simulink model "SPPC"  (R2026a)
settings: Solver=FixedStepDiscrete  StopTime=inf  FixedStep=Ts
model workspace (MATLAB code in the model file):
  | % Defaults for standalone use and code generation, from HPP_parameters.
  | % In HPP.slx the Model block passes p.ctrl.sppc.par as the argument "par".
  | pDefault = HPP_parameters();
  | Ts  = pDefault.ctrl.sppc.Ts;    % [s] fixed sample time
  | par = pDefault.ctrl.sppc.par;   % tunable parameters (model argument)
  | N   = numel(par.share);   % asset instances (fixed per build)
  | clear pDefault
libraries: simulink x5, slpidlib x2, sl_discontinuities x1
Description:
  | SPPC plant controller: WECC REPC_A structure (P control with frequency droop and PI, Q or voltage control with PI, references fed forward), closed loop on the plant feeder into the 33 kV busbar, then dispatch over the N assets by availability. Per unit on the plant rating. Parameters: model argument par (= p.ctrl.sppc.par, from p.pc.sppc).
settings Model: ParameterArgumentNames=par  Creator=kjaer  LastModifiedBy=kjaer

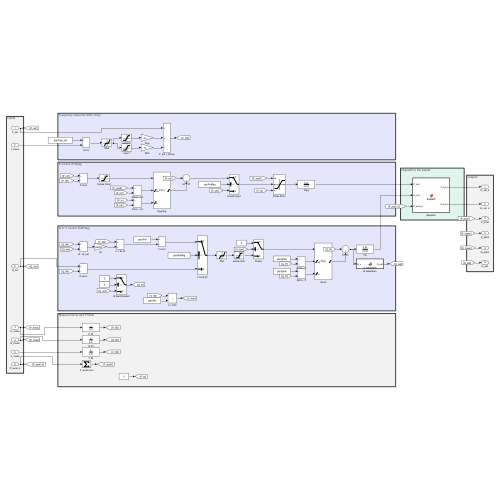
[thumbnail: Simulink's stored preview of the top-level diagram]
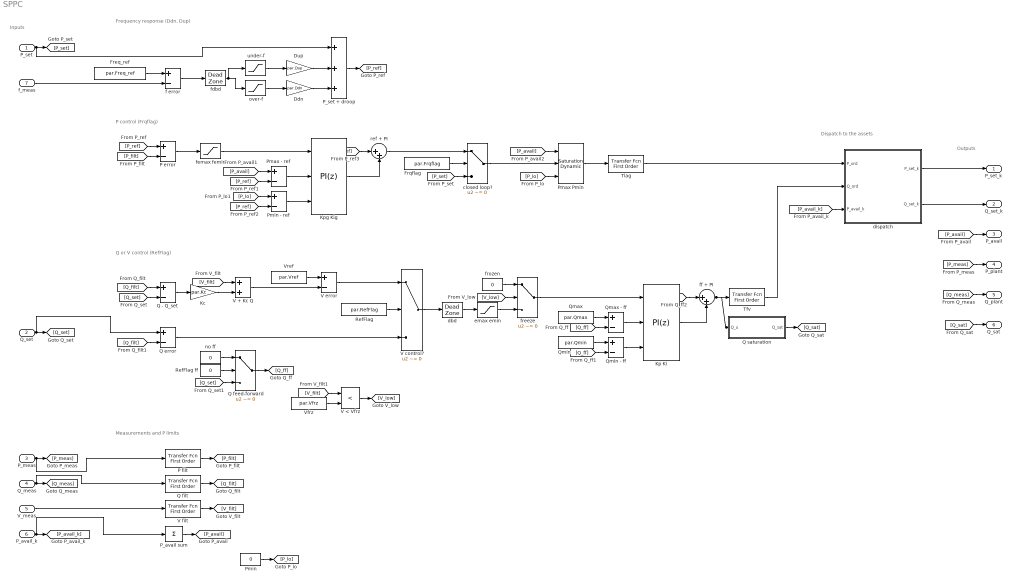
== system SPPC ==
  note: Inputs
  note: Frequency response (Ddn, Dup)
  note: P control (Frqflag)
  note: Q or V control (RefFlag)
  note: Measurements and P limits
  note: Dispatch to the assets
  note: Outputs
  P_set : Inport  OutDataTypeStr=double  PortDimensions=1  SampleTime=Ts
  Q_set : Inport  Port=2  OutDataTypeStr=double  PortDimensions=1  SampleTime=Ts
  P_meas : Inport  Port=3  OutDataTypeStr=double  PortDimensions=1  SampleTime=Ts
  Q_meas : Inport  Port=4  OutDataTypeStr=double  PortDimensions=1  SampleTime=Ts
  V_meas : Inport  Port=5  OutDataTypeStr=double  PortDimensions=1  SampleTime=Ts
  P_avail_k : Inport  Port=6  OutDataTypeStr=double  PortDimensions=N  SampleTime=Ts
  f_meas : Inport  Port=7  OutDataTypeStr=double  PortDimensions=1  SampleTime=Ts
  Ddn : Gain  Gain=par.Ddn
  Dup : Gain  Gain=par.Dup
  Freq_ref : Constant  Value=par.Freq_ref
  Frqflag : Constant  Value=par.Frqflag
  Kc : Gain  Gain=par.Kc
  Kp Ki : slpidlib/PID Controller  Controller=PI  Form=Parallel  TimeDomain=Discrete-time  UseExternalTs=off  SampleTime=-1  IntegratorMethod=Forward Euler  FilterMethod=Forward Euler  ControllerParametersSource=internal  P=par.Kp + par.RefFlag*(par.KpV / (par.Kc + par.dVdQ) - par.Kp)  I=par.Ki + par.RefFlag*(par.KiV / (par.Kc + par.dVdQ) - par.Ki)  UseKiTs=off  D=0  UseExternalDerivativeSource=off  N=100  UseFilter=on  TunerSelectOption=Transfer Function Based (PID Tuner App)  InitialConditionSource=internal  InitialConditionForIntegrator=0  InitialConditionForFilter=0  DifferentiatorICPrevScaledInput=0  ExternalReset=none  TrackingMode=off  Kt=1  LimitOutput=on  SatLimitsSource=external  UpperSaturationLimit=inf  LowerSaturationLimit=-inf  LinearizeAsGain=off  AntiWindupMode=clamping  Kb=1  LimitIntegrator=off  UpperIntegratorSaturationLimit=inf  LowerIntegratorSaturationLimit=-inf  POutMin=[]  POutMax=[]  IOutMin=[]  IOutMax=[]  DOutMin=[]  DOutMax=[]  NOutMin=[]  NOutMax=[]  SumOutMin=[]  SumOutMax=[]  SaturationOutMin=[]  SaturationOutMax=[]  PParamMin=[]  PParamMax=[]  IParamMin=[]  IParamMax=[]  DParamMin=[]  DParamMax=[]  NParamMin=[]  NParamMax=[]  KbParamMin=[]  KbParamMax=[]  KtParamMin=[]  KtParamMax=[]  KbOutMin=[]  KbOutMax=[]  KtOutMin=[]  KtOutMax=[]  IntegratorOutMin=[]  IntegratorOutMax=[]  FilterOutMin=[]  FilterOutMax=[]  SumI1OutMin=[]  SumI1OutMax=[]  SumI2OutMin=[]  SumI2OutMax=[]  SumI3OutMin=[]  SumI3OutMax=[]  SumI4OutMin=[]  SumI4OutMax=[]  SumDOutMin=[]  SumDOutMax=[]  DifferentiatorOutMin=[]  DifferentiatorOutMax=[]  FilterDiffOutCoefMin=[]  FilterDiffOutCoefMax=[]  ReciprocalOutMin=[]  ReciprocalOutMax=[]  SumDenOutMin=[]  SumDenOutMax=[]  SumNumOutMin=[]  SumNumOutMax=[]  DivideOutMin=[]  DivideOutMax=[]  UdiffTsProdOutMin=[]  UdiffTsProdOutMax=[]  NTsProdOutMin=[]  NTsProdOutMax=[]  UintegralTsProdOutMin=[]  UintegralTsProdOutMax=[]  UngainTsProdOutMin=[]  UngainTsProdOutMax=[]  ClampingZeroOutDataTypeStr=Inherit: Inherit via back propagation  ClampingZeroOutMin=[]  ClampingZeroOutMax=[]  FilterDenConstantOutDataTypeStr=Inherit: Inherit via back propagation  FilterDenConstantOutMin=[]  FilterDenConstantOutMax=[]  PCopyOutDataTypeStr=Inherit: Inherit via back propagation  PCopyOutMin=[]  PCopyOutMax=[]  NCopyOutDataTypeStr=Inherit: Inherit via back propagation  NCopyOutMin=[]  NCopyOutMax=[]  IntegratorContinuousStateAttributes=''  IntegratorStateMustResolveToSignalObject=off  IntegratorRTWStateStorageClass=Auto  FilterContinuousStateAttributes=''  FilterStateMustResolveToSignalObject=off  FilterRTWStateStorageClass=Auto  ParallelPVariant=InternalParameters  IdealPVariant=Disabled  IVariant=InternalParameters  DVariant=Disabled  IntegratorVariant=Discrete  SatVariant=External  AWVariant=DiscClampingParallel  PCopyVariant=Disabled  TRVariant=Disabled  FdbkBlocksVariant=Forward  IdealPFdbkVariant=Disabled  SatFdbkVariant=Disabled  DerivativeFilterVariant=Disabled  NVariant=Disabled  NCopyVariant=Disabled_SignalSpec  FilterICVariant=Disabled  IntegratorICVariant=InternalICs  ExternalResetVariant=Disabled  TRSumVariant=Passthrough  SumFdbkVariant=Disabled  SumVariant=Sum_PI  TsampFilterVariant=InternalTs  TsampNgainVariant=Passthrough  TsampIntegralVariant=Disabled_SignalSpec  ExternalSaturationOutDataTypeStr=Inherit: Same as second input  DerivativeSourceVariant=Disabled  PreIntVariant=InternalPreInt
      settings: LibrarySourceBlock=simulink/Discrete/Discrete PID Controller
  Kpg Kig : slpidlib/PID Controller  Controller=PI  Form=Parallel  TimeDomain=Discrete-time  UseExternalTs=off  SampleTime=-1  IntegratorMethod=Forward Euler  FilterMethod=Forward Euler  ControllerParametersSource=internal  P=par.Kpg  I=par.Kig  UseKiTs=off  D=0  UseExternalDerivativeSource=off  N=100  UseFilter=on  TunerSelectOption=Transfer Function Based (PID Tuner App)  InitialConditionSource=internal  InitialConditionForIntegrator=0  InitialConditionForFilter=0  DifferentiatorICPrevScaledInput=0  ExternalReset=none  TrackingMode=off  Kt=1  LimitOutput=on  SatLimitsSource=external  UpperSaturationLimit=inf  LowerSaturationLimit=-inf  LinearizeAsGain=off  AntiWindupMode=clamping  Kb=1  LimitIntegrator=off  UpperIntegratorSaturationLimit=inf  LowerIntegratorSaturationLimit=-inf  POutMin=[]  POutMax=[]  IOutMin=[]  IOutMax=[]  DOutMin=[]  DOutMax=[]  NOutMin=[]  NOutMax=[]  SumOutMin=[]  SumOutMax=[]  SaturationOutMin=[]  SaturationOutMax=[]  PParamMin=[]  PParamMax=[]  IParamMin=[]  IParamMax=[]  DParamMin=[]  DParamMax=[]  NParamMin=[]  NParamMax=[]  KbParamMin=[]  KbParamMax=[]  KtParamMin=[]  KtParamMax=[]  KbOutMin=[]  KbOutMax=[]  KtOutMin=[]  KtOutMax=[]  IntegratorOutMin=[]  IntegratorOutMax=[]  FilterOutMin=[]  FilterOutMax=[]  SumI1OutMin=[]  SumI1OutMax=[]  SumI2OutMin=[]  SumI2OutMax=[]  SumI3OutMin=[]  SumI3OutMax=[]  SumI4OutMin=[]  SumI4OutMax=[]  SumDOutMin=[]  SumDOutMax=[]  DifferentiatorOutMin=[]  DifferentiatorOutMax=[]  FilterDiffOutCoefMin=[]  FilterDiffOutCoefMax=[]  ReciprocalOutMin=[]  ReciprocalOutMax=[]  SumDenOutMin=[]  SumDenOutMax=[]  SumNumOutMin=[]  SumNumOutMax=[]  DivideOutMin=[]  DivideOutMax=[]  UdiffTsProdOutMin=[]  UdiffTsProdOutMax=[]  NTsProdOutMin=[]  NTsProdOutMax=[]  UintegralTsProdOutMin=[]  UintegralTsProdOutMax=[]  UngainTsProdOutMin=[]  UngainTsProdOutMax=[]  ClampingZeroOutDataTypeStr=Inherit: Inherit via back propagation  ClampingZeroOutMin=[]  ClampingZeroOutMax=[]  FilterDenConstantOutDataTypeStr=Inherit: Inherit via back propagation  FilterDenConstantOutMin=[]  FilterDenConstantOutMax=[]  PCopyOutDataTypeStr=Inherit: Inherit via back propagation  PCopyOutMin=[]  PCopyOutMax=[]  NCopyOutDataTypeStr=Inherit: Inherit via back propagation  NCopyOutMin=[]  NCopyOutMax=[]  IntegratorContinuousStateAttributes=''  IntegratorStateMustResolveToSignalObject=off  IntegratorRTWStateStorageClass=Auto  FilterContinuousStateAttributes=''  FilterStateMustResolveToSignalObject=off  FilterRTWStateStorageClass=Auto  ParallelPVariant=InternalParameters  IdealPVariant=Disabled  IVariant=InternalParameters  DVariant=Disabled  IntegratorVariant=Discrete  SatVariant=External  AWVariant=DiscClampingParallel  PCopyVariant=Disabled  TRVariant=Disabled  FdbkBlocksVariant=Forward  IdealPFdbkVariant=Disabled  SatFdbkVariant=Disabled  DerivativeFilterVariant=Disabled  NVariant=Disabled  NCopyVariant=Disabled_SignalSpec  FilterICVariant=Disabled  IntegratorICVariant=InternalICs  ExternalResetVariant=Disabled  TRSumVariant=Passthrough  SumFdbkVariant=Disabled  SumVariant=Sum_PI  TsampFilterVariant=InternalTs  TsampNgainVariant=Passthrough  TsampIntegralVariant=Disabled_SignalSpec  ExternalSaturationOutDataTypeStr=Inherit: Same as second input  DerivativeSourceVariant=Disabled  PreIntVariant=InternalPreInt
      settings: LibrarySourceBlock=simulink/Discrete/Discrete PID Controller
  P error : Sum  Inputs=+-
  P filt : simulink/Discrete/Transfer Fcn First Order  PoleZ=1 - Ts/par.Tp  ICPrevOutput=0  DoSatur=off
  P_avail sum : Sum  Inputs=+
  P_set + droop : Sum  Inputs=+++
  Pmax - ref : Sum  Inputs=+-
  Pmax Pmin : sl_discontinuities/Saturation Dynamic  OutMin=[]  OutMax=[]  OutDataTypeStr=Inherit: Same as second input  OutDataType=fixdt(1, 16)  OutScaling=2^-10  DoSatur=off
      settings: LibrarySourceBlock=|
      | simulink/Discontinuities/Saturation
      | Dynamic
  Pmin : Constant  Value=0
  Pmin - ref : Sum  Inputs=+-
  Q - Q_set : Sum  Inputs=+-
  Q error : Sum  Inputs=+-
  Q feed-forward : Switch  Criteria=u2 ~= 0  SaturateOnIntegerOverflow=off  InputSameDT=off
  Q filt : simulink/Discrete/Transfer Fcn First Order  PoleZ=1 - Ts/par.Tfltr  ICPrevOutput=0  DoSatur=off
  Q saturation : MATLAB Function  TreatAsAtomicUnit=on
  Qmax : Constant  Value=par.Qmax
  Qmax - ff : Sum  Inputs=+-
  Qmin : Constant  Value=par.Qmin
  Qmin - ff : Sum  Inputs=+-
  RefFlag : Constant  Value=par.RefFlag
  RefFlag ff : Constant  Value=0
  Tfv : simulink/Discrete/Transfer Fcn First Order  PoleZ=1 - Ts/par.Tfv  ICPrevOutput=0  DoSatur=off
  Tlag : simulink/Discrete/Transfer Fcn First Order  PoleZ=1 - Ts/par.Tlag  ICPrevOutput=0  DoSatur=off
  V + Kc Q : Sum
  V < Vfrz : RelationalOperator  Operator=<  OutDataTypeStr=boolean  RndMeth=Simplest  InputSameDT=off
  V control? : Switch  Criteria=u2 ~= 0  SaturateOnIntegerOverflow=off  InputSameDT=off
  V error : Sum  Inputs=+-
  V filt : simulink/Discrete/Transfer Fcn First Order  PoleZ=1 - Ts/par.Tfltr  ICPrevOutput=1  DoSatur=off
  Vfrz : Constant  Value=par.Vfrz
  Vref : Constant  Value=par.Vref
  closed loop? : Switch  Criteria=u2 ~= 0  SaturateOnIntegerOverflow=off  InputSameDT=off
  dbd : DeadZone  LowerValue=par.dbd1  UpperValue=par.dbd2
  dispatch : MATLAB Function  TreatAsAtomicUnit=on
  emax emin : Saturate  UpperLimit=par.emax  LowerLimit=par.emin
  f error : Sum  Inputs=+-
  fdbd : DeadZone  LowerValue=par.fdbd1  UpperValue=par.fdbd2
  femax femin : Saturate  UpperLimit=par.femax  LowerLimit=par.femin
  ff + PI : Sum  Inputs=|++
  freeze : Switch  Criteria=u2 ~= 0  SaturateOnIntegerOverflow=off  InputSameDT=off
  frozen : Constant  Value=0
  no ff : Constant  Value=0
  over-f : Saturate  UpperLimit=0  LowerLimit=-inf
  ref + PI : Sum  Inputs=|++
  under-f : Saturate  UpperLimit=inf  LowerLimit=0
  P_set_k : Outport  OutDataTypeStr=double
  Q_set_k : Outport  Port=2  OutDataTypeStr=double
  P_avail : Outport  Port=3  OutDataTypeStr=double
  P_plant : Outport  Port=4  OutDataTypeStr=double
  Q_plant : Outport  Port=5  OutDataTypeStr=double
  Q_sat : Outport  Port=6  OutDataTypeStr=double
  wires:
  P filt/1 -> [P_filt]
  [P_filt] -> P error/2
  P_avail sum/1 -> [P_avail]
  [P_avail] -> P_avail/1
  [P_avail] -> Pmax - ref/1
  [P_avail] -> Pmax Pmin/1
  P_avail_k/1 -> [P_avail_k], P_avail sum/1
  [P_avail_k] -> dispatch/3(P_avail_k)
  P_meas/1 -> [P_meas], P filt/1
  [P_meas] -> P_plant/1
  P_set + droop/1 -> [P_ref]
  [P_ref] -> P error/1
  [P_ref] -> Pmax - ref/2
  [P_ref] -> Pmin - ref/2
  [P_ref] -> ref + PI/1
  P_set/1 -> [P_set], P_set + droop/1
  [P_set] -> closed loop?/3
  Pmin/1 -> [P_lo]
  [P_lo] -> Pmax Pmin/3
  [P_lo] -> Pmin - ref/1
  Q feed-forward/1 -> [Q_ff]
  [Q_ff] -> Qmax - ff/2
  [Q_ff] -> Qmin - ff/2
  [Q_ff] -> ff + PI/1
  Q filt/1 -> [Q_filt]
  [Q_filt] -> Q - Q_set/1
  [Q_filt] -> Q error/2
  Q saturation/1(Q_sat) -> [Q_sat]
  [Q_sat] -> Q_sat/1
  Q_meas/1 -> [Q_meas], Q filt/1
  [Q_meas] -> Q_plant/1
  Q_set/1 -> [Q_set], Q error/1
  [Q_set] -> Q - Q_set/2
  [Q_set] -> Q feed-forward/3
  V < Vfrz/1 -> [V_low]
  [V_low] -> freeze/2
  V filt/1 -> [V_filt]
  [V_filt] -> V + Kc Q/1
  [V_filt] -> V < Vfrz/1
  Ddn/1 -> P_set + droop/3
  Dup/1 -> P_set + droop/2
  Freq_ref/1 -> f error/1
  Frqflag/1 -> closed loop?/2
  Kc/1 -> V + Kc Q/2
  Kp Ki/1 -> ff + PI/2
  Kpg Kig/1 -> ref + PI/2
  P error/1 -> femax femin/1
  Pmax - ref/1 -> Kpg Kig/2
  Pmax Pmin/1 -> Tlag/1
  Pmin - ref/1 -> Kpg Kig/3
  Q - Q_set/1 -> Kc/1
  Q error/1 -> V control?/3
  Qmax - ff/1 -> Kp Ki/2
  Qmax/1 -> Qmax - ff/1
  Qmin - ff/1 -> Kp Ki/3
  Qmin/1 -> Qmin - ff/1
  RefFlag ff/1 -> Q feed-forward/2
  RefFlag/1 -> V control?/2
  Tfv/1 -> dispatch/2(Q_ord)
  Tlag/1 -> dispatch/1(P_ord)
  V + Kc Q/1 -> V error/2
  V control?/1 -> dbd/1
  V error/1 -> V control?/1
  V_meas/1 -> V filt/1
  Vfrz/1 -> V < Vfrz/2
  Vref/1 -> V error/1
  closed loop?/1 -> Pmax Pmin/2
  dbd/1 -> emax emin/1
  dispatch/1(P_set_k) -> P_set_k/1
  dispatch/2(Q_set_k) -> Q_set_k/1
  emax emin/1 -> freeze/3
  f error/1 -> fdbd/1
  f_meas/1 -> f error/2
  fdbd/1 -> over-f/1, under-f/1
  femax femin/1 -> Kpg Kig/1
  ff + PI/1 -> Q saturation/1(Q_u), Tfv/1
  freeze/1 -> Kp Ki/1
  frozen/1 -> freeze/1
  no ff/1 -> Q feed-forward/1
  over-f/1 -> Ddn/1
  ref + PI/1 -> closed loop?/1
  under-f/1 -> Dup/1

== matlab function SPPC/dispatch ==
  data: P_ord input; P_set_k output; Q_ord input; P_avail_k input; Q_set_k output; par parameter
function [P_set_k, Q_set_k] = dispatch(P_ord, Q_ord, P_avail_k, par)
%#codegen
% Split the plant P and Q orders over the assets in proportion to
% their availability (equal shares if nothing is available).
a = P_avail_k;
s = sum(a);
if s > 1e-6
    w = a / s;
else
    w = par.share;
end
P_set_k = P_ord * w;
Q_set_k = Q_ord * par.share;   % Q by rating share (also with no availability)
end

== matlab function SPPC/Q saturation ==
  data: Q_u input; Q_sat output; par parameter
function Q_sat  = q_saturation(Q_u, par)
%#codegen
tol = 1e-4;
Q_sat = double(Q_u >= par.Qmax - tol) - double(Q_u <= par.Qmin + tol);
end
